simulink model "WarehouseFleetSim"  (R2024b)
settings: Solver=ode4  StartTime=0.0  StopTime=inf  FixedStep=0.02  RelTol=1e-3
StopFcn:
  | try, fleetVisionStep('close'); catch, end; try, phase3('stopped'); catch, end
model workspace (MAT data in the model file):
  HomePose1 = [-20 7.3 0]
  HomePose2 = [-20 3.6 0]
  HomePose3 = [-20 11 0]
  HomePose4 = [-24.5 3.6 0]
  HomePose5 = [-24.5 7.3 0]
  HomePose6 = [-24.5 11 0]
  Zero = 0
  gen3 : robotics.RigidBodyTree (value not decoded)
  qStow = [0; 0; 0.261799387799; 3.14159265359; -2.26892802759; 0; 0.959931088597; 1.57079632679]
undefined symbols (not defined in the file or in its folder): Actor, setupFleetScene, Sim3dSensor, World
libraries: sim3dlib x128, sim3dcameralib x7, robotmobilelib x6, robotsim3dlib x6
(part 3 of 4)

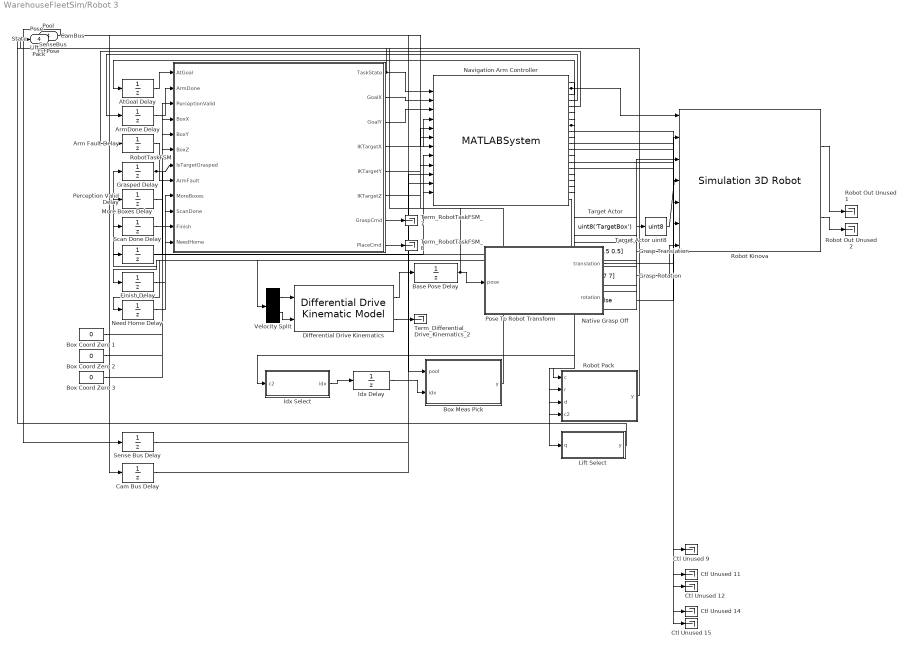
== system WarehouseFleetSim/Robot 3 ==
  Pool : Inport
  EstPose : Inport  Port=2
  SenseBus : Inport  Port=3
  CamBus : Inport  Port=4
  Arm Fault Delay : UnitDelay  InitialCondition=false  SampleTime=0.02  HasFrameUpgradeWarning=on
  ArmDone Delay : UnitDelay  InitialCondition=false  SampleTime=0.02  HasFrameUpgradeWarning=on
  AtGoal Delay : UnitDelay  InitialCondition=false  SampleTime=0.02  HasFrameUpgradeWarning=on
  Base Pose Delay : UnitDelay  InitialCondition=HomePose3  SampleTime=0.02  HasFrameUpgradeWarning=on
  Box Coord Zero 1 : Constant  Value=0  OutDataTypeStr=double
  Box Coord Zero 2 : Constant  Value=0  OutDataTypeStr=double
  Box Coord Zero 3 : Constant  Value=0  OutDataTypeStr=double
  Box Meas Pick : MATLAB Function  TreatAsAtomicUnit=on
  Cam Bus Delay : UnitDelay  InitialCondition=zeros(1,8)  SampleTime=0.02  HasFrameUpgradeWarning=on
  Ctl Unused {9,11..12,14..15} (5 alike) : Terminator
  Differential Drive Kinematics : robotmobilelib/Differential Drive Kinematic Model  VehicleInputs=Vehicle Speed & Heading Angular Velocity  WheelRadius=0.05  WheelSpeedRange=[-inf inf]  TrackWidth=0.2  InitialState=HomePose3  SimulateUsing=Interpreted execution
  Finish Delay : UnitDelay  InitialCondition=false  SampleTime=0.02  HasFrameUpgradeWarning=on
  Grasp Rotation : Constant  Value=[7 7 7]
  Grasp Translation : Constant  Value=[0.5 0.5 0.5]
  Grasped Delay : UnitDelay  InitialCondition=false  SampleTime=0.02  HasFrameUpgradeWarning=on
  Idx Delay : UnitDelay  SampleTime=0.02  HasFrameUpgradeWarning=on
  Idx Select : MATLAB Function  TreatAsAtomicUnit=on
  Lift Select : MATLAB Function  TreatAsAtomicUnit=on
  More Boxes Delay : UnitDelay  InitialCondition=false  SampleTime=0.02  HasFrameUpgradeWarning=on
  Native Grasp Off : Constant  Value=false  OutDataTypeStr=boolean
  Navigation Arm Controller : MATLABSystem  System=WarehouseRobotControlSystemV23  SampleTime=0.02  RobotId=3  SimulateUsing=Interpreted execution
      mask Type: WarehouseRobotControlSystemV23
      mask Display:
      | disp('WarehouseRobotControlSystemV23');
      | port_label('input',1,'state');
      | port_label('input',2,'~');
      | port_label('input',3,'~');
      | port_label('input',4,'~');
      | port_label('input',5,'~');
      | port_label('input',6,'~');
      | port_label('input',7,'basePose');
      | port_label('input',8,'isTargetGrasped');
      | port_label('input',9,'boxMeas');
      | port_label('input',10,'senseBus');
      | port_label('input',11,'camBus');
      | port_label('input',12,'truePose');
      | port_label('output',1,'velocity');
      | port_label('output',2,'config');
      | port_label('output',3,'atGoal');
      | port_label('output',4,'armDone');
      | port_label('output',5,'armFault');
      | port_label('output',6,'vacuum');
      | port_label('output',7,'c1');
      | port_label('output',8,'c2');
      | port_label('output',9,'c3');
      | port_label('output',10,'r1');
      | port_label('output',11,'r2');
      | port_label('output',12,'r3');
      | port_label('output',13,'d1');
      | port_label('output',14,'d2');
      | port_label('output',15,'d3');
      | port_label('output',16,'percValid');
      | port_label('output',17,'moreBoxes');
      | port_label('output',18,'scanDone');
      | port_label('output',19,'finish');
      | port_label('output',20,'needHome');
  Need Home Delay : UnitDelay  InitialCondition=false  SampleTime=0.02  HasFrameUpgradeWarning=on
  Perception Valid Delay : UnitDelay  InitialCondition=false  SampleTime=0.02  HasFrameUpgradeWarning=on
  Pose To Robot Transform : MATLAB Function  TreatAsAtomicUnit=on
  Robot Kinova : robotsim3dlib/Simulation 3D Robot  Priority=2  actorInputType=RigidBodyTree Object  RigidBodyTree=gen3  ActorName=Ro3Kinova  existActorChekBox=off  initialTrans=[0 0 0]  initialRot=[0 0 0]  initialConfig=qStow  EndEffector=ToolTip  eeOffsetInpChekBox=off  eeTargetTrans=[-0.04 0 0.245]  eeTargetRot=[0 1.2217 3.1416]  enableRegionGraspChekBox=on  regionGraspInpChekBox=on  eeTargTransDiff=[0.2 0.2 0.2]  eeTargRotDiff=[0 0 0]  inpConfEnbVal=on  inpGraspEnbVal=on  inpTransEnbVal=on  outConfEnbVal=on  outGraspEnbVal=on  outTransEnbVal=off  SampleTime=0.02  ActorType=SimulinkVehicle  ID=C  aMode=6  ActorTag=Ro3Kinova  Mesh=RigidBodyTree
  Robot Out Unused 1 : Terminator
  Robot Out Unused 2 : Terminator
  Robot Pack : MATLAB Function  TreatAsAtomicUnit=on
  RobotTaskFSM : Stateflow chart  TreatAsAtomicUnit=on
  Scan Done Delay : UnitDelay  InitialCondition=false  SampleTime=0.02  HasFrameUpgradeWarning=on
  Sense Bus Delay : UnitDelay  InitialCondition=zeros(1,8)  SampleTime=0.02  HasFrameUpgradeWarning=on
  Target Actor : Constant  Value=uint8('TargetBox')  OutDataTypeStr=uint8
  Target Actor uint8 : DataTypeConversion  OutDataTypeStr=uint8  SaturateOnIntegerOverflow=off  RndMeth=Floor
  Term_Differential_Drive_Kinematics_2 : Terminator
  Term_RobotTaskFSM_7 : Terminator
  Term_RobotTaskFSM_8 : Terminator
  Velocity Split : Demux  Outputs=2
  Pose : Outport
  Pack : Outport  Port=2
  Lift : Outport  Port=3
  State : Outport  Port=4
  wires:
  Navigation Arm Controller/3 -> AtGoal Delay/1
  AtGoal Delay/1 -> RobotTaskFSM/1(AtGoal)
  Navigation Arm Controller/4 -> ArmDone Delay/1
  ArmDone Delay/1 -> RobotTaskFSM/2(ArmDone)
  Navigation Arm Controller/5 -> Arm Fault Delay/1
  Arm Fault Delay/1 -> RobotTaskFSM/8(ArmFault)
  Navigation Arm Controller/6 -> Grasped Delay/1
  Grasped Delay/1 -> RobotTaskFSM/7(IsTargetGrasped), Navigation Arm Controller/8
  Navigation Arm Controller/16 -> Perception Valid Delay/1
  Perception Valid Delay/1 -> RobotTaskFSM/3(PerceptionValid)
  Navigation Arm Controller/17 -> More Boxes Delay/1
  More Boxes Delay/1 -> RobotTaskFSM/9(MoreBoxes)
  Navigation Arm Controller/18 -> Scan Done Delay/1
  Scan Done Delay/1 -> RobotTaskFSM/10(ScanDone)
  Navigation Arm Controller/19 -> Finish Delay/1
  Finish Delay/1 -> RobotTaskFSM/11(Finish)
  Navigation Arm Controller/20 -> Need Home Delay/1
  Need Home Delay/1 -> RobotTaskFSM/12(NeedHome)
  Box Coord Zero 1/1 -> RobotTaskFSM/4(BoxX)
  Box Coord Zero 2/1 -> RobotTaskFSM/5(BoxY)
  Box Coord Zero 3/1 -> RobotTaskFSM/6(BoxZ)
  RobotTaskFSM/1(TaskState) -> Navigation Arm Controller/1, State/1
  RobotTaskFSM/2(GoalX) -> Navigation Arm Controller/2
  RobotTaskFSM/3(GoalY) -> Navigation Arm Controller/3
  RobotTaskFSM/4(IKTargetX) -> Navigation Arm Controller/4
  RobotTaskFSM/5(IKTargetY) -> Navigation Arm Controller/5
  RobotTaskFSM/6(IKTargetZ) -> Navigation Arm Controller/6
  EstPose/1 -> Navigation Arm Controller/7
  SenseBus/1 -> Sense Bus Delay/1
  Sense Bus Delay/1 -> Navigation Arm Controller/10
  CamBus/1 -> Cam Bus Delay/1
  Cam Bus Delay/1 -> Navigation Arm Controller/11
  Base Pose Delay/1 -> Navigation Arm Controller/12, Pose/1, Pose To Robot Transform/1(pose)
  Navigation Arm Controller/8 -> Idx Select/1(c2), Robot Pack/4(c2)
  Idx Select/1(idx) -> Idx Delay/1
  Idx Delay/1 -> Box Meas Pick/2(idx)
  Pool/1 -> Box Meas Pick/1(pool)
  Box Meas Pick/1(y) -> Navigation Arm Controller/9
  Navigation Arm Controller/7 -> Robot Pack/1(c)
  Navigation Arm Controller/10 -> Robot Pack/2(r)
  Navigation Arm Controller/13 -> Robot Pack/3(d)
  Robot Pack/1(y) -> Pack/1
  Navigation Arm Controller/2 -> Lift Select/1(q), Robot Kinova/1
  Lift Select/1(y) -> Lift/1
  Navigation Arm Controller/9 -> Ctl Unused 9/1
  Navigation Arm Controller/11 -> Ctl Unused 11/1
  Navigation Arm Controller/12 -> Ctl Unused 12/1
  Navigation Arm Controller/14 -> Ctl Unused 14/1
  Navigation Arm Controller/15 -> Ctl Unused 15/1
  Navigation Arm Controller/1 -> Velocity Split/1
  Velocity Split/1 -> Differential Drive Kinematics/1
  Velocity Split/2 -> Differential Drive Kinematics/2
  Differential Drive Kinematics/1 -> Base Pose Delay/1
  Target Actor/1 -> Target Actor uint8/1
  Pose To Robot Transform/1(translation) -> Robot Kinova/2
  Pose To Robot Transform/2(rotation) -> Robot Kinova/3
  Target Actor uint8/1 -> Robot Kinova/4
  Native Grasp Off/1 -> Robot Kinova/5
  Grasp Translation/1 -> Robot Kinova/6
  Grasp Rotation/1 -> Robot Kinova/7
  Robot Kinova/1 -> Robot Out Unused 1/1
  Robot Kinova/2 -> Robot Out Unused 2/1
  Differential Drive Kinematics/2 -> Term_Differential_Drive_Kinematics_2/1
  RobotTaskFSM/7(GraspCmd) -> Term_RobotTaskFSM_7/1
  RobotTaskFSM/8(PlaceCmd) -> Term_RobotTaskFSM_8/1

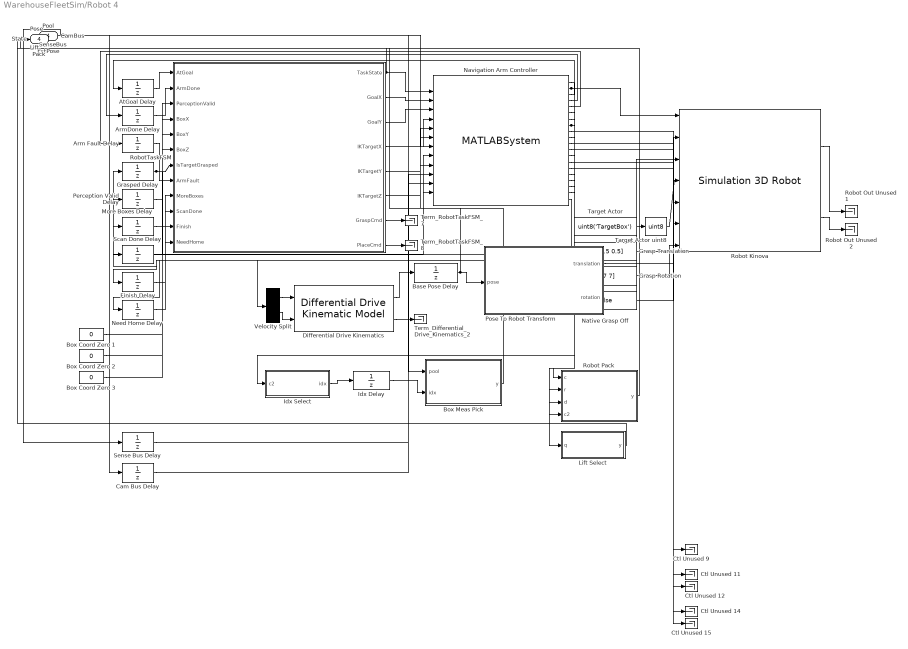
== system WarehouseFleetSim/Robot 4 ==
  Pool : Inport
  EstPose : Inport  Port=2
  SenseBus : Inport  Port=3
  CamBus : Inport  Port=4
  Arm Fault Delay : UnitDelay  InitialCondition=false  SampleTime=0.02  HasFrameUpgradeWarning=on
  ArmDone Delay : UnitDelay  InitialCondition=false  SampleTime=0.02  HasFrameUpgradeWarning=on
  AtGoal Delay : UnitDelay  InitialCondition=false  SampleTime=0.02  HasFrameUpgradeWarning=on
  Base Pose Delay : UnitDelay  InitialCondition=HomePose4  SampleTime=0.02  HasFrameUpgradeWarning=on
  Box Coord Zero 1 : Constant  Value=0  OutDataTypeStr=double
  Box Coord Zero 2 : Constant  Value=0  OutDataTypeStr=double
  Box Coord Zero 3 : Constant  Value=0  OutDataTypeStr=double
  Box Meas Pick : MATLAB Function  TreatAsAtomicUnit=on
  Cam Bus Delay : UnitDelay  InitialCondition=zeros(1,8)  SampleTime=0.02  HasFrameUpgradeWarning=on
  Ctl Unused {9,11..12,14..15} (5 alike) : Terminator
  Differential Drive Kinematics : robotmobilelib/Differential Drive Kinematic Model  VehicleInputs=Vehicle Speed & Heading Angular Velocity  WheelRadius=0.05  WheelSpeedRange=[-inf inf]  TrackWidth=0.2  InitialState=HomePose4  SimulateUsing=Interpreted execution
  Finish Delay : UnitDelay  InitialCondition=false  SampleTime=0.02  HasFrameUpgradeWarning=on
  Grasp Rotation : Constant  Value=[7 7 7]
  Grasp Translation : Constant  Value=[0.5 0.5 0.5]
  Grasped Delay : UnitDelay  InitialCondition=false  SampleTime=0.02  HasFrameUpgradeWarning=on
  Idx Delay : UnitDelay  SampleTime=0.02  HasFrameUpgradeWarning=on
  Idx Select : MATLAB Function  TreatAsAtomicUnit=on
  Lift Select : MATLAB Function  TreatAsAtomicUnit=on
  More Boxes Delay : UnitDelay  InitialCondition=false  SampleTime=0.02  HasFrameUpgradeWarning=on
  Native Grasp Off : Constant  Value=false  OutDataTypeStr=boolean
  Navigation Arm Controller : MATLABSystem  System=WarehouseRobotControlSystemV23  SampleTime=0.02  RobotId=4  SimulateUsing=Interpreted execution
      mask Type: WarehouseRobotControlSystemV23
      mask Display:
      | disp('WarehouseRobotControlSystemV23');
      | port_label('input',1,'state');
      | port_label('input',2,'~');
      | port_label('input',3,'~');
      | port_label('input',4,'~');
      | port_label('input',5,'~');
      | port_label('input',6,'~');
      | port_label('input',7,'basePose');
      | port_label('input',8,'isTargetGrasped');
      | port_label('input',9,'boxMeas');
      | port_label('input',10,'senseBus');
      | port_label('input',11,'camBus');
      | port_label('input',12,'truePose');
      | port_label('output',1,'velocity');
      | port_label('output',2,'config');
      | port_label('output',3,'atGoal');
      | port_label('output',4,'armDone');
      | port_label('output',5,'armFault');
      | port_label('output',6,'vacuum');
      | port_label('output',7,'c1');
      | port_label('output',8,'c2');
      | port_label('output',9,'c3');
      | port_label('output',10,'r1');
      | port_label('output',11,'r2');
      | port_label('output',12,'r3');
      | port_label('output',13,'d1');
      | port_label('output',14,'d2');
      | port_label('output',15,'d3');
      | port_label('output',16,'percValid');
      | port_label('output',17,'moreBoxes');
      | port_label('output',18,'scanDone');
      | port_label('output',19,'finish');
      | port_label('output',20,'needHome');
  Need Home Delay : UnitDelay  InitialCondition=false  SampleTime=0.02  HasFrameUpgradeWarning=on
  Perception Valid Delay : UnitDelay  InitialCondition=false  SampleTime=0.02  HasFrameUpgradeWarning=on
  Pose To Robot Transform : MATLAB Function  TreatAsAtomicUnit=on
  Robot Kinova : robotsim3dlib/Simulation 3D Robot  Priority=2  actorInputType=RigidBodyTree Object  RigidBodyTree=gen3  ActorName=Ro4Kinova  existActorChekBox=off  initialTrans=[0 0 0]  initialRot=[0 0 0]  initialConfig=qStow  EndEffector=ToolTip  eeOffsetInpChekBox=off  eeTargetTrans=[-0.04 0 0.245]  eeTargetRot=[0 1.2217 3.1416]  enableRegionGraspChekBox=on  regionGraspInpChekBox=on  eeTargTransDiff=[0.2 0.2 0.2]  eeTargRotDiff=[0 0 0]  inpConfEnbVal=on  inpGraspEnbVal=on  inpTransEnbVal=on  outConfEnbVal=on  outGraspEnbVal=on  outTransEnbVal=off  SampleTime=0.02  ActorType=SimulinkVehicle  ID=C  aMode=6  ActorTag=Ro4Kinova  Mesh=RigidBodyTree
  Robot Out Unused 1 : Terminator
  Robot Out Unused 2 : Terminator
  Robot Pack : MATLAB Function  TreatAsAtomicUnit=on
  RobotTaskFSM : Stateflow chart  TreatAsAtomicUnit=on
  Scan Done Delay : UnitDelay  InitialCondition=false  SampleTime=0.02  HasFrameUpgradeWarning=on
  Sense Bus Delay : UnitDelay  InitialCondition=zeros(1,8)  SampleTime=0.02  HasFrameUpgradeWarning=on
  Target Actor : Constant  Value=uint8('TargetBox')  OutDataTypeStr=uint8
  Target Actor uint8 : DataTypeConversion  OutDataTypeStr=uint8  SaturateOnIntegerOverflow=off  RndMeth=Floor
  Term_Differential_Drive_Kinematics_2 : Terminator
  Term_RobotTaskFSM_7 : Terminator
  Term_RobotTaskFSM_8 : Terminator
  Velocity Split : Demux  Outputs=2
  Pose : Outport
  Pack : Outport  Port=2
  Lift : Outport  Port=3
  State : Outport  Port=4
  wires:
  Navigation Arm Controller/3 -> AtGoal Delay/1
  AtGoal Delay/1 -> RobotTaskFSM/1(AtGoal)
  Navigation Arm Controller/4 -> ArmDone Delay/1
  ArmDone Delay/1 -> RobotTaskFSM/2(ArmDone)
  Navigation Arm Controller/5 -> Arm Fault Delay/1
  Arm Fault Delay/1 -> RobotTaskFSM/8(ArmFault)
  Navigation Arm Controller/6 -> Grasped Delay/1
  Grasped Delay/1 -> RobotTaskFSM/7(IsTargetGrasped), Navigation Arm Controller/8
  Navigation Arm Controller/16 -> Perception Valid Delay/1
  Perception Valid Delay/1 -> RobotTaskFSM/3(PerceptionValid)
  Navigation Arm Controller/17 -> More Boxes Delay/1
  More Boxes Delay/1 -> RobotTaskFSM/9(MoreBoxes)
  Navigation Arm Controller/18 -> Scan Done Delay/1
  Scan Done Delay/1 -> RobotTaskFSM/10(ScanDone)
  Navigation Arm Controller/19 -> Finish Delay/1
  Finish Delay/1 -> RobotTaskFSM/11(Finish)
  Navigation Arm Controller/20 -> Need Home Delay/1
  Need Home Delay/1 -> RobotTaskFSM/12(NeedHome)
  Box Coord Zero 1/1 -> RobotTaskFSM/4(BoxX)
  Box Coord Zero 2/1 -> RobotTaskFSM/5(BoxY)
  Box Coord Zero 3/1 -> RobotTaskFSM/6(BoxZ)
  RobotTaskFSM/1(TaskState) -> Navigation Arm Controller/1, State/1
  RobotTaskFSM/2(GoalX) -> Navigation Arm Controller/2
  RobotTaskFSM/3(GoalY) -> Navigation Arm Controller/3
  RobotTaskFSM/4(IKTargetX) -> Navigation Arm Controller/4
  RobotTaskFSM/5(IKTargetY) -> Navigation Arm Controller/5
  RobotTaskFSM/6(IKTargetZ) -> Navigation Arm Controller/6
  EstPose/1 -> Navigation Arm Controller/7
  SenseBus/1 -> Sense Bus Delay/1
  Sense Bus Delay/1 -> Navigation Arm Controller/10
  CamBus/1 -> Cam Bus Delay/1
  Cam Bus Delay/1 -> Navigation Arm Controller/11
  Base Pose Delay/1 -> Navigation Arm Controller/12, Pose/1, Pose To Robot Transform/1(pose)
  Navigation Arm Controller/8 -> Idx Select/1(c2), Robot Pack/4(c2)
  Idx Select/1(idx) -> Idx Delay/1
  Idx Delay/1 -> Box Meas Pick/2(idx)
  Pool/1 -> Box Meas Pick/1(pool)
  Box Meas Pick/1(y) -> Navigation Arm Controller/9
  Navigation Arm Controller/7 -> Robot Pack/1(c)
  Navigation Arm Controller/10 -> Robot Pack/2(r)
  Navigation Arm Controller/13 -> Robot Pack/3(d)
  Robot Pack/1(y) -> Pack/1
  Navigation Arm Controller/2 -> Lift Select/1(q), Robot Kinova/1
  Lift Select/1(y) -> Lift/1
  Navigation Arm Controller/9 -> Ctl Unused 9/1
  Navigation Arm Controller/11 -> Ctl Unused 11/1
  Navigation Arm Controller/12 -> Ctl Unused 12/1
  Navigation Arm Controller/14 -> Ctl Unused 14/1
  Navigation Arm Controller/15 -> Ctl Unused 15/1
  Navigation Arm Controller/1 -> Velocity Split/1
  Velocity Split/1 -> Differential Drive Kinematics/1
  Velocity Split/2 -> Differential Drive Kinematics/2
  Differential Drive Kinematics/1 -> Base Pose Delay/1
  Target Actor/1 -> Target Actor uint8/1
  Pose To Robot Transform/1(translation) -> Robot Kinova/2
  Pose To Robot Transform/2(rotation) -> Robot Kinova/3
  Target Actor uint8/1 -> Robot Kinova/4
  Native Grasp Off/1 -> Robot Kinova/5
  Grasp Translation/1 -> Robot Kinova/6
  Grasp Rotation/1 -> Robot Kinova/7
  Robot Kinova/1 -> Robot Out Unused 1/1
  Robot Kinova/2 -> Robot Out Unused 2/1
  Differential Drive Kinematics/2 -> Term_Differential_Drive_Kinematics_2/1
  RobotTaskFSM/7(GraspCmd) -> Term_RobotTaskFSM_7/1
  RobotTaskFSM/8(PlaceCmd) -> Term_RobotTaskFSM_8/1

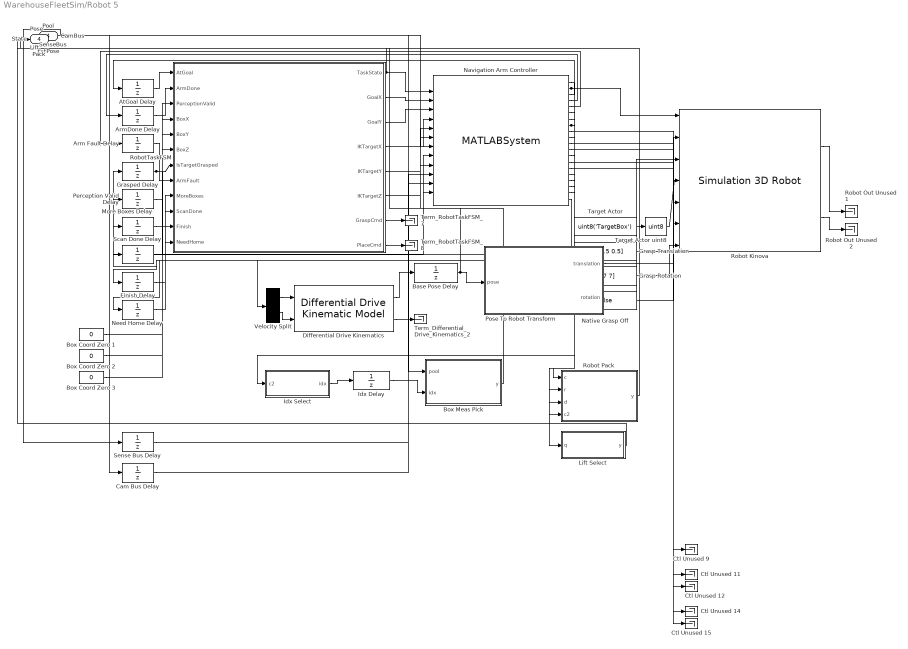
== system WarehouseFleetSim/Robot 5 ==
  Pool : Inport
  EstPose : Inport  Port=2
  SenseBus : Inport  Port=3
  CamBus : Inport  Port=4
  Arm Fault Delay : UnitDelay  InitialCondition=false  SampleTime=0.02  HasFrameUpgradeWarning=on
  ArmDone Delay : UnitDelay  InitialCondition=false  SampleTime=0.02  HasFrameUpgradeWarning=on
  AtGoal Delay : UnitDelay  InitialCondition=false  SampleTime=0.02  HasFrameUpgradeWarning=on
  Base Pose Delay : UnitDelay  InitialCondition=HomePose5  SampleTime=0.02  HasFrameUpgradeWarning=on
  Box Coord Zero 1 : Constant  Value=0  OutDataTypeStr=double
  Box Coord Zero 2 : Constant  Value=0  OutDataTypeStr=double
  Box Coord Zero 3 : Constant  Value=0  OutDataTypeStr=double
  Box Meas Pick : MATLAB Function  TreatAsAtomicUnit=on
  Cam Bus Delay : UnitDelay  InitialCondition=zeros(1,8)  SampleTime=0.02  HasFrameUpgradeWarning=on
  Ctl Unused {9,11..12,14..15} (5 alike) : Terminator
  Differential Drive Kinematics : robotmobilelib/Differential Drive Kinematic Model  VehicleInputs=Vehicle Speed & Heading Angular Velocity  WheelRadius=0.05  WheelSpeedRange=[-inf inf]  TrackWidth=0.2  InitialState=HomePose5  SimulateUsing=Interpreted execution
  Finish Delay : UnitDelay  InitialCondition=false  SampleTime=0.02  HasFrameUpgradeWarning=on
  Grasp Rotation : Constant  Value=[7 7 7]
  Grasp Translation : Constant  Value=[0.5 0.5 0.5]
  Grasped Delay : UnitDelay  InitialCondition=false  SampleTime=0.02  HasFrameUpgradeWarning=on
  Idx Delay : UnitDelay  SampleTime=0.02  HasFrameUpgradeWarning=on
  Idx Select : MATLAB Function  TreatAsAtomicUnit=on
  Lift Select : MATLAB Function  TreatAsAtomicUnit=on
  More Boxes Delay : UnitDelay  InitialCondition=false  SampleTime=0.02  HasFrameUpgradeWarning=on
  Native Grasp Off : Constant  Value=false  OutDataTypeStr=boolean
  Navigation Arm Controller : MATLABSystem  System=WarehouseRobotControlSystemV23  SampleTime=0.02  RobotId=5  SimulateUsing=Interpreted execution
      mask Type: WarehouseRobotControlSystemV23
      mask Display:
      | disp('WarehouseRobotControlSystemV23');
      | port_label('input',1,'state');
      | port_label('input',2,'~');
      | port_label('input',3,'~');
      | port_label('input',4,'~');
      | port_label('input',5,'~');
      | port_label('input',6,'~');
      | port_label('input',7,'basePose');
      | port_label('input',8,'isTargetGrasped');
      | port_label('input',9,'boxMeas');
      | port_label('input',10,'senseBus');
      | port_label('input',11,'camBus');
      | port_label('input',12,'truePose');
      | port_label('output',1,'velocity');
      | port_label('output',2,'config');
      | port_label('output',3,'atGoal');
      | port_label('output',4,'armDone');
      | port_label('output',5,'armFault');
      | port_label('output',6,'vacuum');
      | port_label('output',7,'c1');
      | port_label('output',8,'c2');
      | port_label('output',9,'c3');
      | port_label('output',10,'r1');
      | port_label('output',11,'r2');
      | port_label('output',12,'r3');
      | port_label('output',13,'d1');
      | port_label('output',14,'d2');
      | port_label('output',15,'d3');
      | port_label('output',16,'percValid');
      | port_label('output',17,'moreBoxes');
      | port_label('output',18,'scanDone');
      | port_label('output',19,'finish');
      | port_label('output',20,'needHome');
  Need Home Delay : UnitDelay  InitialCondition=false  SampleTime=0.02  HasFrameUpgradeWarning=on
  Perception Valid Delay : UnitDelay  InitialCondition=false  SampleTime=0.02  HasFrameUpgradeWarning=on
  Pose To Robot Transform : MATLAB Function  TreatAsAtomicUnit=on
  Robot Kinova : robotsim3dlib/Simulation 3D Robot  Priority=2  actorInputType=RigidBodyTree Object  RigidBodyTree=gen3  ActorName=Ro5Kinova  existActorChekBox=off  initialTrans=[0 0 0]  initialRot=[0 0 0]  initialConfig=qStow  EndEffector=ToolTip  eeOffsetInpChekBox=off  eeTargetTrans=[-0.04 0 0.245]  eeTargetRot=[0 1.2217 3.1416]  enableRegionGraspChekBox=on  regionGraspInpChekBox=on  eeTargTransDiff=[0.2 0.2 0.2]  eeTargRotDiff=[0 0 0]  inpConfEnbVal=on  inpGraspEnbVal=on  inpTransEnbVal=on  outConfEnbVal=on  outGraspEnbVal=on  outTransEnbVal=off  SampleTime=0.02  ActorType=SimulinkVehicle  ID=C  aMode=6  ActorTag=Ro5Kinova  Mesh=RigidBodyTree
  Robot Out Unused 1 : Terminator
  Robot Out Unused 2 : Terminator
  Robot Pack : MATLAB Function  TreatAsAtomicUnit=on
  RobotTaskFSM : Stateflow chart  TreatAsAtomicUnit=on
  Scan Done Delay : UnitDelay  InitialCondition=false  SampleTime=0.02  HasFrameUpgradeWarning=on
  Sense Bus Delay : UnitDelay  InitialCondition=zeros(1,8)  SampleTime=0.02  HasFrameUpgradeWarning=on
  Target Actor : Constant  Value=uint8('TargetBox')  OutDataTypeStr=uint8
  Target Actor uint8 : DataTypeConversion  OutDataTypeStr=uint8  SaturateOnIntegerOverflow=off  RndMeth=Floor
  Term_Differential_Drive_Kinematics_2 : Terminator
  Term_RobotTaskFSM_7 : Terminator
  Term_RobotTaskFSM_8 : Terminator
  Velocity Split : Demux  Outputs=2
  Pose : Outport
  Pack : Outport  Port=2
  Lift : Outport  Port=3
  State : Outport  Port=4
  wires:
  Navigation Arm Controller/3 -> AtGoal Delay/1
  AtGoal Delay/1 -> RobotTaskFSM/1(AtGoal)
  Navigation Arm Controller/4 -> ArmDone Delay/1
  ArmDone Delay/1 -> RobotTaskFSM/2(ArmDone)
  Navigation Arm Controller/5 -> Arm Fault Delay/1
  Arm Fault Delay/1 -> RobotTaskFSM/8(ArmFault)
  Navigation Arm Controller/6 -> Grasped Delay/1
  Grasped Delay/1 -> RobotTaskFSM/7(IsTargetGrasped), Navigation Arm Controller/8
  Navigation Arm Controller/16 -> Perception Valid Delay/1
  Perception Valid Delay/1 -> RobotTaskFSM/3(PerceptionValid)
  Navigation Arm Controller/17 -> More Boxes Delay/1
  More Boxes Delay/1 -> RobotTaskFSM/9(MoreBoxes)
  Navigation Arm Controller/18 -> Scan Done Delay/1
  Scan Done Delay/1 -> RobotTaskFSM/10(ScanDone)
  Navigation Arm Controller/19 -> Finish Delay/1
  Finish Delay/1 -> RobotTaskFSM/11(Finish)
  Navigation Arm Controller/20 -> Need Home Delay/1
  Need Home Delay/1 -> RobotTaskFSM/12(NeedHome)
  Box Coord Zero 1/1 -> RobotTaskFSM/4(BoxX)
  Box Coord Zero 2/1 -> RobotTaskFSM/5(BoxY)
  Box Coord Zero 3/1 -> RobotTaskFSM/6(BoxZ)
  RobotTaskFSM/1(TaskState) -> Navigation Arm Controller/1, State/1
  RobotTaskFSM/2(GoalX) -> Navigation Arm Controller/2
  RobotTaskFSM/3(GoalY) -> Navigation Arm Controller/3
  RobotTaskFSM/4(IKTargetX) -> Navigation Arm Controller/4
  RobotTaskFSM/5(IKTargetY) -> Navigation Arm Controller/5
  RobotTaskFSM/6(IKTargetZ) -> Navigation Arm Controller/6
  EstPose/1 -> Navigation Arm Controller/7
  SenseBus/1 -> Sense Bus Delay/1
  Sense Bus Delay/1 -> Navigation Arm Controller/10
  CamBus/1 -> Cam Bus Delay/1
  Cam Bus Delay/1 -> Navigation Arm Controller/11
  Base Pose Delay/1 -> Navigation Arm Controller/12, Pose/1, Pose To Robot Transform/1(pose)
  Navigation Arm Controller/8 -> Idx Select/1(c2), Robot Pack/4(c2)
  Idx Select/1(idx) -> Idx Delay/1
  Idx Delay/1 -> Box Meas Pick/2(idx)
  Pool/1 -> Box Meas Pick/1(pool)
  Box Meas Pick/1(y) -> Navigation Arm Controller/9
  Navigation Arm Controller/7 -> Robot Pack/1(c)
  Navigation Arm Controller/10 -> Robot Pack/2(r)
  Navigation Arm Controller/13 -> Robot Pack/3(d)
  Robot Pack/1(y) -> Pack/1
  Navigation Arm Controller/2 -> Lift Select/1(q), Robot Kinova/1
  Lift Select/1(y) -> Lift/1
  Navigation Arm Controller/9 -> Ctl Unused 9/1
  Navigation Arm Controller/11 -> Ctl Unused 11/1
  Navigation Arm Controller/12 -> Ctl Unused 12/1
  Navigation Arm Controller/14 -> Ctl Unused 14/1
  Navigation Arm Controller/15 -> Ctl Unused 15/1
  Navigation Arm Controller/1 -> Velocity Split/1
  Velocity Split/1 -> Differential Drive Kinematics/1
  Velocity Split/2 -> Differential Drive Kinematics/2
  Differential Drive Kinematics/1 -> Base Pose Delay/1
  Target Actor/1 -> Target Actor uint8/1
  Pose To Robot Transform/1(translation) -> Robot Kinova/2
  Pose To Robot Transform/2(rotation) -> Robot Kinova/3
  Target Actor uint8/1 -> Robot Kinova/4
  Native Grasp Off/1 -> Robot Kinova/5
  Grasp Translation/1 -> Robot Kinova/6
  Grasp Rotation/1 -> Robot Kinova/7
  Robot Kinova/1 -> Robot Out Unused 1/1
  Robot Kinova/2 -> Robot Out Unused 2/1
  Differential Drive Kinematics/2 -> Term_Differential_Drive_Kinematics_2/1
  RobotTaskFSM/7(GraspCmd) -> Term_RobotTaskFSM_7/1
  RobotTaskFSM/8(PlaceCmd) -> Term_RobotTaskFSM_8/1

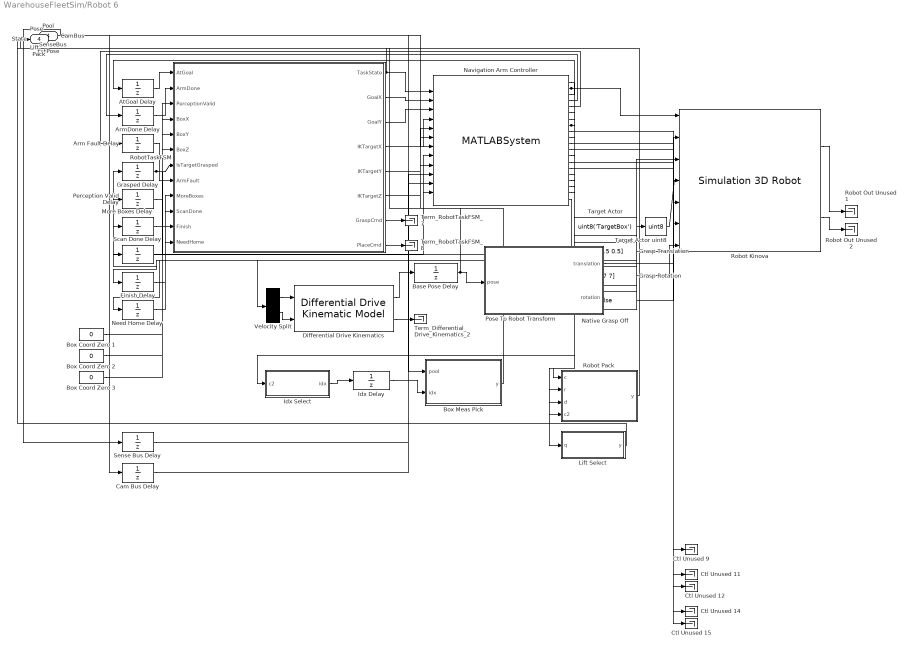
== system WarehouseFleetSim/Robot 6 ==
  Pool : Inport
  EstPose : Inport  Port=2
  SenseBus : Inport  Port=3
  CamBus : Inport  Port=4
  Arm Fault Delay : UnitDelay  InitialCondition=false  SampleTime=0.02  HasFrameUpgradeWarning=on
  ArmDone Delay : UnitDelay  InitialCondition=false  SampleTime=0.02  HasFrameUpgradeWarning=on
  AtGoal Delay : UnitDelay  InitialCondition=false  SampleTime=0.02  HasFrameUpgradeWarning=on
  Base Pose Delay : UnitDelay  InitialCondition=HomePose6  SampleTime=0.02  HasFrameUpgradeWarning=on
  Box Coord Zero 1 : Constant  Value=0  OutDataTypeStr=double
  Box Coord Zero 2 : Constant  Value=0  OutDataTypeStr=double
  Box Coord Zero 3 : Constant  Value=0  OutDataTypeStr=double
  Box Meas Pick : MATLAB Function  TreatAsAtomicUnit=on
  Cam Bus Delay : UnitDelay  InitialCondition=zeros(1,8)  SampleTime=0.02  HasFrameUpgradeWarning=on
  Ctl Unused {9,11..12,14..15} (5 alike) : Terminator
  Differential Drive Kinematics : robotmobilelib/Differential Drive Kinematic Model  VehicleInputs=Vehicle Speed & Heading Angular Velocity  WheelRadius=0.05  WheelSpeedRange=[-inf inf]  TrackWidth=0.2  InitialState=HomePose6  SimulateUsing=Interpreted execution
  Finish Delay : UnitDelay  InitialCondition=false  SampleTime=0.02  HasFrameUpgradeWarning=on
  Grasp Rotation : Constant  Value=[7 7 7]
  Grasp Translation : Constant  Value=[0.5 0.5 0.5]
  Grasped Delay : UnitDelay  InitialCondition=false  SampleTime=0.02  HasFrameUpgradeWarning=on
  Idx Delay : UnitDelay  SampleTime=0.02  HasFrameUpgradeWarning=on
  Idx Select : MATLAB Function  TreatAsAtomicUnit=on
  Lift Select : MATLAB Function  TreatAsAtomicUnit=on
  More Boxes Delay : UnitDelay  InitialCondition=false  SampleTime=0.02  HasFrameUpgradeWarning=on
  Native Grasp Off : Constant  Value=false  OutDataTypeStr=boolean
  Navigation Arm Controller : MATLABSystem  System=WarehouseRobotControlSystemV23  SampleTime=0.02  RobotId=6  SimulateUsing=Interpreted execution
      mask Type: WarehouseRobotControlSystemV23
      mask Display:
      | disp('WarehouseRobotControlSystemV23');
      | port_label('input',1,'state');
      | port_label('input',2,'~');
      | port_label('input',3,'~');
      | port_label('input',4,'~');
      | port_label('input',5,'~');
      | port_label('input',6,'~');
      | port_label('input',7,'basePose');
      | port_label('input',8,'isTargetGrasped');
      | port_label('input',9,'boxMeas');
      | port_label('input',10,'senseBus');
      | port_label('input',11,'camBus');
      | port_label('input',12,'truePose');
      | port_label('output',1,'velocity');
      | port_label('output',2,'config');
      | port_label('output',3,'atGoal');
      | port_label('output',4,'armDone');
      | port_label('output',5,'armFault');
      | port_label('output',6,'vacuum');
      | port_label('output',7,'c1');
      | port_label('output',8,'c2');
      | port_label('output',9,'c3');
      | port_label('output',10,'r1');
      | port_label('output',11,'r2');
      | port_label('output',12,'r3');
      | port_label('output',13,'d1');
      | port_label('output',14,'d2');
      | port_label('output',15,'d3');
      | port_label('output',16,'percValid');
      | port_label('output',17,'moreBoxes');
      | port_label('output',18,'scanDone');
      | port_label('output',19,'finish');
      | port_label('output',20,'needHome');
  Need Home Delay : UnitDelay  InitialCondition=false  SampleTime=0.02  HasFrameUpgradeWarning=on
  Perception Valid Delay : UnitDelay  InitialCondition=false  SampleTime=0.02  HasFrameUpgradeWarning=on
  Pose To Robot Transform : MATLAB Function  TreatAsAtomicUnit=on
  Robot Kinova : robotsim3dlib/Simulation 3D Robot  Priority=2  actorInputType=RigidBodyTree Object  RigidBodyTree=gen3  ActorName=Ro6Kinova  existActorChekBox=off  initialTrans=[0 0 0]  initialRot=[0 0 0]  initialConfig=qStow  EndEffector=ToolTip  eeOffsetInpChekBox=off  eeTargetTrans=[-0.04 0 0.245]  eeTargetRot=[0 1.2217 3.1416]  enableRegionGraspChekBox=on  regionGraspInpChekBox=on  eeTargTransDiff=[0.2 0.2 0.2]  eeTargRotDiff=[0 0 0]  inpConfEnbVal=on  inpGraspEnbVal=on  inpTransEnbVal=on  outConfEnbVal=on  outGraspEnbVal=on  outTransEnbVal=off  SampleTime=0.02  ActorType=SimulinkVehicle  ID=C  aMode=6  ActorTag=Ro6Kinova  Mesh=RigidBodyTree
  Robot Out Unused 1 : Terminator
  Robot Out Unused 2 : Terminator
  Robot Pack : MATLAB Function  TreatAsAtomicUnit=on
  RobotTaskFSM : Stateflow chart  TreatAsAtomicUnit=on
  Scan Done Delay : UnitDelay  InitialCondition=false  SampleTime=0.02  HasFrameUpgradeWarning=on
  Sense Bus Delay : UnitDelay  InitialCondition=zeros(1,8)  SampleTime=0.02  HasFrameUpgradeWarning=on
  Target Actor : Constant  Value=uint8('TargetBox')  OutDataTypeStr=uint8
  Target Actor uint8 : DataTypeConversion  OutDataTypeStr=uint8  SaturateOnIntegerOverflow=off  RndMeth=Floor
  Term_Differential_Drive_Kinematics_2 : Terminator
  Term_RobotTaskFSM_7 : Terminator
  Term_RobotTaskFSM_8 : Terminator
  Velocity Split : Demux  Outputs=2
  Pose : Outport
  Pack : Outport  Port=2
  Lift : Outport  Port=3
  State : Outport  Port=4
  wires:
  Navigation Arm Controller/3 -> AtGoal Delay/1
  AtGoal Delay/1 -> RobotTaskFSM/1(AtGoal)
  Navigation Arm Controller/4 -> ArmDone Delay/1
  ArmDone Delay/1 -> RobotTaskFSM/2(ArmDone)
  Navigation Arm Controller/5 -> Arm Fault Delay/1
  Arm Fault Delay/1 -> RobotTaskFSM/8(ArmFault)
  Navigation Arm Controller/6 -> Grasped Delay/1
  Grasped Delay/1 -> RobotTaskFSM/7(IsTargetGrasped), Navigation Arm Controller/8
  Navigation Arm Controller/16 -> Perception Valid Delay/1
  Perception Valid Delay/1 -> RobotTaskFSM/3(PerceptionValid)
  Navigation Arm Controller/17 -> More Boxes Delay/1
  More Boxes Delay/1 -> RobotTaskFSM/9(MoreBoxes)
  Navigation Arm Controller/18 -> Scan Done Delay/1
  Scan Done Delay/1 -> RobotTaskFSM/10(ScanDone)
  Navigation Arm Controller/19 -> Finish Delay/1
  Finish Delay/1 -> RobotTaskFSM/11(Finish)
  Navigation Arm Controller/20 -> Need Home Delay/1
  Need Home Delay/1 -> RobotTaskFSM/12(NeedHome)
  Box Coord Zero 1/1 -> RobotTaskFSM/4(BoxX)
  Box Coord Zero 2/1 -> RobotTaskFSM/5(BoxY)
  Box Coord Zero 3/1 -> RobotTaskFSM/6(BoxZ)
  RobotTaskFSM/1(TaskState) -> Navigation Arm Controller/1, State/1
  RobotTaskFSM/2(GoalX) -> Navigation Arm Controller/2
  RobotTaskFSM/3(GoalY) -> Navigation Arm Controller/3
  RobotTaskFSM/4(IKTargetX) -> Navigation Arm Controller/4
  RobotTaskFSM/5(IKTargetY) -> Navigation Arm Controller/5
  RobotTaskFSM/6(IKTargetZ) -> Navigation Arm Controller/6
  EstPose/1 -> Navigation Arm Controller/7
  SenseBus/1 -> Sense Bus Delay/1
  Sense Bus Delay/1 -> Navigation Arm Controller/10
  CamBus/1 -> Cam Bus Delay/1
  Cam Bus Delay/1 -> Navigation Arm Controller/11
  Base Pose Delay/1 -> Navigation Arm Controller/12, Pose/1, Pose To Robot Transform/1(pose)
  Navigation Arm Controller/8 -> Idx Select/1(c2), Robot Pack/4(c2)
  Idx Select/1(idx) -> Idx Delay/1
  Idx Delay/1 -> Box Meas Pick/2(idx)
  Pool/1 -> Box Meas Pick/1(pool)
  Box Meas Pick/1(y) -> Navigation Arm Controller/9
  Navigation Arm Controller/7 -> Robot Pack/1(c)
  Navigation Arm Controller/10 -> Robot Pack/2(r)
  Navigation Arm Controller/13 -> Robot Pack/3(d)
  Robot Pack/1(y) -> Pack/1
  Navigation Arm Controller/2 -> Lift Select/1(q), Robot Kinova/1
  Lift Select/1(y) -> Lift/1
  Navigation Arm Controller/9 -> Ctl Unused 9/1
  Navigation Arm Controller/11 -> Ctl Unused 11/1
  Navigation Arm Controller/12 -> Ctl Unused 12/1
  Navigation Arm Controller/14 -> Ctl Unused 14/1
  Navigation Arm Controller/15 -> Ctl Unused 15/1
  Navigation Arm Controller/1 -> Velocity Split/1
  Velocity Split/1 -> Differential Drive Kinematics/1
  Velocity Split/2 -> Differential Drive Kinematics/2
  Differential Drive Kinematics/1 -> Base Pose Delay/1
  Target Actor/1 -> Target Actor uint8/1
  Pose To Robot Transform/1(translation) -> Robot Kinova/2
  Pose To Robot Transform/2(rotation) -> Robot Kinova/3
  Target Actor uint8/1 -> Robot Kinova/4
  Native Grasp Off/1 -> Robot Kinova/5
  Grasp Translation/1 -> Robot Kinova/6
  Grasp Rotation/1 -> Robot Kinova/7
  Robot Kinova/1 -> Robot Out Unused 1/1
  Robot Kinova/2 -> Robot Out Unused 2/1
  Differential Drive Kinematics/2 -> Term_Differential_Drive_Kinematics_2/1
  RobotTaskFSM/7(GraspCmd) -> Term_RobotTaskFSM_7/1
  RobotTaskFSM/8(PlaceCmd) -> Term_RobotTaskFSM_8/1

== stateflow chart WarehouseFleetSim/Robot 1/RobotTaskFSM ==
  settings: updateMethod=DISCRETE  sampleTime=0.02
  state IDLE
    en: TaskState=uint8(0); GoalX=-20.0000; GoalY=7.3000; GraspCmd=false; PlaceCmd=false;
  state NAV_TO_STAGING
    en: TaskState=uint8(1); GoalX=15.5000; GoalY=46.0556; GraspCmd=false; PlaceCmd=false;
  state DOCK_SHELF
    en: TaskState=uint8(10); GoalX=14.1900; GoalY=46.0556; IKTargetX=BoxX; IKTargetY=BoxY; IKTargetZ=BoxZ; GraspCmd=false; PlaceCmd=false;
  state ARM_EXTEND
    en: TaskState=uint8(2); IKTargetX=BoxX; IKTargetY=BoxY; IKTargetZ=BoxZ; GraspCmd=false;
  state GRASP
    en: TaskState=uint8(3); GraspCmd=true; PlaceCmd=false;
  state ARM_RETRACT
    en: TaskState=uint8(4); GraspCmd=true; PlaceCmd=false;
  state NAV_TO_TABLE
    en: TaskState=uint8(5); GoalX=18.5000; GoalY=65.1000; GraspCmd=true;
  state ARM_PLACE
    en: TaskState=uint8(6); IKTargetX=18.5000; IKTargetY=65.9700; IKTargetZ=1.0700; GraspCmd=true;
  state RELEASE
    en: TaskState=uint8(8); GraspCmd=false; PlaceCmd=true;
  state ARM_STOW
    en: TaskState=uint8(9); GraspCmd=false; PlaceCmd=false;
  state RETURN_HOME
    en: TaskState=uint8(7); GoalX=-20.0000; GoalY=7.3000; GraspCmd=false;
  state FAULT_HOLD
    en: TaskState=uint8(11); GraspCmd=false; PlaceCmd=false;
  state MISSION_DONE
    en: TaskState=uint8(12); GoalX=-20.0000; GoalY=7.3000; GraspCmd=false; PlaceCmd=false;
  NAV_TO_STAGING -> IDLE [order 2] : [AtGoal && ScanDone && ~PerceptionValid]
  RETURN_HOME -> IDLE : [AtGoal || MoreBoxes]
  (default) -> IDLE
  GRASP -> ARM_RETRACT [order 2] : [ArmDone && IsTargetGrasped]
  DOCK_SHELF -> FAULT_HOLD [order 2] : [ArmFault]
  ARM_EXTEND -> FAULT_HOLD [order 1] : [ArmFault]
  GRASP -> FAULT_HOLD [order 1] : [ArmFault]
  IDLE -> NAV_TO_STAGING [order 1] : after(1,sec)[MoreBoxes]
  NAV_TO_STAGING -> DOCK_SHELF [order 1] : [AtGoal && ScanDone && PerceptionValid]
  DOCK_SHELF -> ARM_EXTEND [order 1] : [AtGoal && ArmDone]
  ARM_EXTEND -> GRASP [order 2] : [ArmDone]
  IDLE -> MISSION_DONE [order 3] : after(2,sec)[~MoreBoxes && Finish && ~NeedHome]
  IDLE -> RETURN_HOME [order 2] : after(1,sec)[~MoreBoxes && NeedHome]
  FAULT_HOLD -> ARM_RETRACT [order 1] : [~ArmFault && IsTargetGrasped]
  ARM_RETRACT -> NAV_TO_TABLE [order 2] : [ArmDone]
  ARM_STOW -> RETURN_HOME : [ArmDone]
  NAV_TO_TABLE -> ARM_PLACE : [AtGoal]
  ARM_PLACE -> FAULT_HOLD [order 1] : [ArmFault]
  ARM_PLACE -> RELEASE [order 2] : [ArmDone]
  FAULT_HOLD -> ARM_STOW [order 2] : [~ArmFault && ~IsTargetGrasped]
  RELEASE -> ARM_STOW [order 1] : [~IsTargetGrasped]
  RELEASE -> ARM_STOW [order 2] : after(1,sec)
  ARM_RETRACT -> FAULT_HOLD [order 1] : [ArmFault]
  data: AtGoal input boolean; ArmDone input boolean; PerceptionValid input boolean; BoxX input double; BoxY input double; BoxZ input double; IsTargetGrasped input boolean; ArmFault input boolean; MoreBoxes input boolean; ScanDone input boolean; Finish input boolean; NeedHome input boolean; TaskState output uint8; GoalX output double; GoalY output double; IKTargetX output double; IKTargetY output double; IKTargetZ output double; GraspCmd output boolean; PlaceCmd output boolean

== matlab function WarehouseFleetSim/Robot 1/Box Meas Pick ==
  data: pool input; y output; idx input
function y = fcn(pool,idx)
y = zeros(1,9); i = round(idx);
if i>=1 && i<=54, y(1:3) = pool(3*i-2:3*i); end

== matlab function WarehouseFleetSim/Robot 1/Robot Pack ==
  data: c input; y output; r input; d input; c2 input
function y = fcn(c,r,d,c2)
y = [c r double(d) c2(1)];

== matlab function WarehouseFleetSim/Robot 1/Lift Select ==
  data: q input; y output
function y = fcn(q)
y = q(1);

== matlab function WarehouseFleetSim/Robot 1/Pose To Robot Transform ==
  data: pose input; translation output; rotation output
function [translation,rotation] = fcn(pose)
translation = [pose(1), pose(2), 0];
rotation = [pose(3), 0, 0];

== stateflow chart WarehouseFleetSim/Robot 2/RobotTaskFSM ==
  settings: updateMethod=DISCRETE  sampleTime=0.02
  state IDLE
    en: TaskState=uint8(0); GoalX=-20.0000; GoalY=3.6000; GraspCmd=false; PlaceCmd=false;
  state NAV_TO_STAGING
    en: TaskState=uint8(1); GoalX=15.5000; GoalY=46.0556; GraspCmd=false; PlaceCmd=false;
  state DOCK_SHELF
    en: TaskState=uint8(10); GoalX=14.1900; GoalY=46.0556; IKTargetX=BoxX; IKTargetY=BoxY; IKTargetZ=BoxZ; GraspCmd=false; PlaceCmd=false;
  state ARM_EXTEND
    en: TaskState=uint8(2); IKTargetX=BoxX; IKTargetY=BoxY; IKTargetZ=BoxZ; GraspCmd=false;
  state GRASP
    en: TaskState=uint8(3); GraspCmd=true; PlaceCmd=false;
  state ARM_RETRACT
    en: TaskState=uint8(4); GraspCmd=true; PlaceCmd=false;
  state NAV_TO_TABLE
    en: TaskState=uint8(5); GoalX=18.5000; GoalY=65.1000; GraspCmd=true;
  state ARM_PLACE
    en: TaskState=uint8(6); IKTargetX=18.5000; IKTargetY=65.9700; IKTargetZ=1.0700; GraspCmd=true;
  state RELEASE
    en: TaskState=uint8(8); GraspCmd=false; PlaceCmd=true;
  state ARM_STOW
    en: TaskState=uint8(9); GraspCmd=false; PlaceCmd=false;
  state RETURN_HOME
    en: TaskState=uint8(7); GoalX=-20.0000; GoalY=3.6000; GraspCmd=false;
  state FAULT_HOLD
    en: TaskState=uint8(11); GraspCmd=false; PlaceCmd=false;
  state MISSION_DONE
    en: TaskState=uint8(12); GoalX=-20.0000; GoalY=3.6000; GraspCmd=false; PlaceCmd=false;
  NAV_TO_STAGING -> IDLE [order 2] : [AtGoal && ScanDone && ~PerceptionValid]
  RETURN_HOME -> IDLE : [AtGoal || MoreBoxes]
  (default) -> IDLE
  GRASP -> ARM_RETRACT [order 2] : [ArmDone && IsTargetGrasped]
  DOCK_SHELF -> FAULT_HOLD [order 2] : [ArmFault]
  ARM_EXTEND -> FAULT_HOLD [order 1] : [ArmFault]
  GRASP -> FAULT_HOLD [order 1] : [ArmFault]
  IDLE -> NAV_TO_STAGING [order 1] : after(1,sec)[MoreBoxes]
  NAV_TO_STAGING -> DOCK_SHELF [order 1] : [AtGoal && ScanDone && PerceptionValid]
  DOCK_SHELF -> ARM_EXTEND [order 1] : [AtGoal && ArmDone]
  ARM_EXTEND -> GRASP [order 2] : [ArmDone]
  IDLE -> MISSION_DONE [order 3] : after(2,sec)[~MoreBoxes && Finish && ~NeedHome]
  IDLE -> RETURN_HOME [order 2] : after(1,sec)[~MoreBoxes && NeedHome]
  FAULT_HOLD -> ARM_RETRACT [order 1] : [~ArmFault && IsTargetGrasped]
  ARM_RETRACT -> NAV_TO_TABLE [order 2] : [ArmDone]
  ARM_STOW -> RETURN_HOME : [ArmDone]
  NAV_TO_TABLE -> ARM_PLACE : [AtGoal]
  ARM_PLACE -> FAULT_HOLD [order 1] : [ArmFault]
  ARM_PLACE -> RELEASE [order 2] : [ArmDone]
  FAULT_HOLD -> ARM_STOW [order 2] : [~ArmFault && ~IsTargetGrasped]
  RELEASE -> ARM_STOW [order 1] : [~IsTargetGrasped]
  RELEASE -> ARM_STOW [order 2] : after(1,sec)
  ARM_RETRACT -> FAULT_HOLD [order 1] : [ArmFault]
  data: AtGoal input boolean; ArmDone input boolean; PerceptionValid input boolean; BoxX input double; BoxY input double; BoxZ input double; IsTargetGrasped input boolean; ArmFault input boolean; MoreBoxes input boolean; ScanDone input boolean; Finish input boolean; NeedHome input boolean; TaskState output uint8; GoalX output double; GoalY output double; IKTargetX output double; IKTargetY output double; IKTargetZ output double; GraspCmd output boolean; PlaceCmd output boolean

== matlab function WarehouseFleetSim/Robot 2/Idx Select ==
  data: c2 input; idx output
function idx = fcn(c2)
idx = c2(1);

== matlab function WarehouseFleetSim/Robot 2/Box Meas Pick ==
  data: pool input; y output; idx input
function y = fcn(pool,idx)
y = zeros(1,9); i = round(idx);
if i>=1 && i<=54, y(1:3) = pool(3*i-2:3*i); end

== matlab function WarehouseFleetSim/Robot 2/Robot Pack ==
  data: c input; y output; r input; d input; c2 input
function y = fcn(c,r,d,c2)
y = [c r double(d) c2(1)];

== matlab function WarehouseFleetSim/Robot 2/Lift Select ==
  data: q input; y output
function y = fcn(q)
y = q(1);

== matlab function WarehouseFleetSim/Robot 2/Pose To Robot Transform ==
  data: pose input; translation output; rotation output
function [translation,rotation] = fcn(pose)
translation = [pose(1), pose(2), 0];
rotation = [pose(3), 0, 0];

== stateflow chart WarehouseFleetSim/Robot 3/RobotTaskFSM ==
  settings: updateMethod=DISCRETE  sampleTime=0.02
  state IDLE
    en: TaskState=uint8(0); GoalX=-20.0000; GoalY=11.0000; GraspCmd=false; PlaceCmd=false;
  state NAV_TO_STAGING
    en: TaskState=uint8(1); GoalX=15.5000; GoalY=46.0556; GraspCmd=false; PlaceCmd=false;
  state DOCK_SHELF
    en: TaskState=uint8(10); GoalX=14.1900; GoalY=46.0556; IKTargetX=BoxX; IKTargetY=BoxY; IKTargetZ=BoxZ; GraspCmd=false; PlaceCmd=false;
  state ARM_EXTEND
    en: TaskState=uint8(2); IKTargetX=BoxX; IKTargetY=BoxY; IKTargetZ=BoxZ; GraspCmd=false;
  state GRASP
    en: TaskState=uint8(3); GraspCmd=true; PlaceCmd=false;
  state ARM_RETRACT
    en: TaskState=uint8(4); GraspCmd=true; PlaceCmd=false;
  state NAV_TO_TABLE
    en: TaskState=uint8(5); GoalX=18.5000; GoalY=65.1000; GraspCmd=true;
  state ARM_PLACE
    en: TaskState=uint8(6); IKTargetX=18.5000; IKTargetY=65.9700; IKTargetZ=1.0700; GraspCmd=true;
  state RELEASE
    en: TaskState=uint8(8); GraspCmd=false; PlaceCmd=true;
  state ARM_STOW
    en: TaskState=uint8(9); GraspCmd=false; PlaceCmd=false;
  state RETURN_HOME
    en: TaskState=uint8(7); GoalX=-20.0000; GoalY=11.0000; GraspCmd=false;
  state FAULT_HOLD
    en: TaskState=uint8(11); GraspCmd=false; PlaceCmd=false;
  state MISSION_DONE
    en: TaskState=uint8(12); GoalX=-20.0000; GoalY=11.0000; GraspCmd=false; PlaceCmd=false;
  NAV_TO_STAGING -> IDLE [order 2] : [AtGoal && ScanDone && ~PerceptionValid]
  RETURN_HOME -> IDLE : [AtGoal || MoreBoxes]
  (default) -> IDLE
  GRASP -> ARM_RETRACT [order 2] : [ArmDone && IsTargetGrasped]
  DOCK_SHELF -> FAULT_HOLD [order 2] : [ArmFault]
  ARM_EXTEND -> FAULT_HOLD [order 1] : [ArmFault]
  GRASP -> FAULT_HOLD [order 1] : [ArmFault]
  IDLE -> NAV_TO_STAGING [order 1] : after(1,sec)[MoreBoxes]
  NAV_TO_STAGING -> DOCK_SHELF [order 1] : [AtGoal && ScanDone && PerceptionValid]
  DOCK_SHELF -> ARM_EXTEND [order 1] : [AtGoal && ArmDone]
  ARM_EXTEND -> GRASP [order 2] : [ArmDone]
  IDLE -> MISSION_DONE [order 3] : after(2,sec)[~MoreBoxes && Finish && ~NeedHome]
  IDLE -> RETURN_HOME [order 2] : after(1,sec)[~MoreBoxes && NeedHome]
  FAULT_HOLD -> ARM_RETRACT [order 1] : [~ArmFault && IsTargetGrasped]
  ARM_RETRACT -> NAV_TO_TABLE [order 2] : [ArmDone]
  ARM_STOW -> RETURN_HOME : [ArmDone]
  NAV_TO_TABLE -> ARM_PLACE : [AtGoal]
  ARM_PLACE -> FAULT_HOLD [order 1] : [ArmFault]
  ARM_PLACE -> RELEASE [order 2] : [ArmDone]
  FAULT_HOLD -> ARM_STOW [order 2] : [~ArmFault && ~IsTargetGrasped]
  RELEASE -> ARM_STOW [order 1] : [~IsTargetGrasped]
  RELEASE -> ARM_STOW [order 2] : after(1,sec)
  ARM_RETRACT -> FAULT_HOLD [order 1] : [ArmFault]
  data: AtGoal input boolean; ArmDone input boolean; PerceptionValid input boolean; BoxX input double; BoxY input double; BoxZ input double; IsTargetGrasped input boolean; ArmFault input boolean; MoreBoxes input boolean; ScanDone input boolean; Finish input boolean; NeedHome input boolean; TaskState output uint8; GoalX output double; GoalY output double; IKTargetX output double; IKTargetY output double; IKTargetZ output double; GraspCmd output boolean; PlaceCmd output boolean

== matlab function WarehouseFleetSim/Robot 3/Idx Select ==
  data: c2 input; idx output
function idx = fcn(c2)
idx = c2(1);

== matlab function WarehouseFleetSim/Robot 3/Box Meas Pick ==
  data: pool input; y output; idx input
function y = fcn(pool,idx)
y = zeros(1,9); i = round(idx);
if i>=1 && i<=54, y(1:3) = pool(3*i-2:3*i); end

== matlab function WarehouseFleetSim/Robot 3/Robot Pack ==
  data: c input; y output; r input; d input; c2 input
function y = fcn(c,r,d,c2)
y = [c r double(d) c2(1)];

== matlab function WarehouseFleetSim/Robot 3/Lift Select ==
  data: q input; y output
function y = fcn(q)
y = q(1);

== matlab function WarehouseFleetSim/Robot 3/Pose To Robot Transform ==
  data: pose input; translation output; rotation output
function [translation,rotation] = fcn(pose)
translation = [pose(1), pose(2), 0];
rotation = [pose(3), 0, 0];

== stateflow chart WarehouseFleetSim/Robot 4/RobotTaskFSM ==
  settings: updateMethod=DISCRETE  sampleTime=0.02
  state IDLE
    en: TaskState=uint8(0); GoalX=-24.5000; GoalY=3.6000; GraspCmd=false; PlaceCmd=false;
  state NAV_TO_STAGING
    en: TaskState=uint8(1); GoalX=15.5000; GoalY=46.0556; GraspCmd=false; PlaceCmd=false;
  state DOCK_SHELF
    en: TaskState=uint8(10); GoalX=14.1900; GoalY=46.0556; IKTargetX=BoxX; IKTargetY=BoxY; IKTargetZ=BoxZ; GraspCmd=false; PlaceCmd=false;
  state ARM_EXTEND
    en: TaskState=uint8(2); IKTargetX=BoxX; IKTargetY=BoxY; IKTargetZ=BoxZ; GraspCmd=false;
  state GRASP
    en: TaskState=uint8(3); GraspCmd=true; PlaceCmd=false;
  state ARM_RETRACT
    en: TaskState=uint8(4); GraspCmd=true; PlaceCmd=false;
  state NAV_TO_TABLE
    en: TaskState=uint8(5); GoalX=18.5000; GoalY=65.1000; GraspCmd=true;
  state ARM_PLACE
    en: TaskState=uint8(6); IKTargetX=18.5000; IKTargetY=65.9700; IKTargetZ=1.0700; GraspCmd=true;
  state RELEASE
    en: TaskState=uint8(8); GraspCmd=false; PlaceCmd=true;
  state ARM_STOW
    en: TaskState=uint8(9); GraspCmd=false; PlaceCmd=false;
  state RETURN_HOME
    en: TaskState=uint8(7); GoalX=-24.5000; GoalY=3.6000; GraspCmd=false;
  state FAULT_HOLD
    en: TaskState=uint8(11); GraspCmd=false; PlaceCmd=false;
  state MISSION_DONE
    en: TaskState=uint8(12); GoalX=-24.5000; GoalY=3.6000; GraspCmd=false; PlaceCmd=false;
  NAV_TO_STAGING -> IDLE [order 2] : [AtGoal && ScanDone && ~PerceptionValid]
  RETURN_HOME -> IDLE : [AtGoal || MoreBoxes]
  (default) -> IDLE
  GRASP -> ARM_RETRACT [order 2] : [ArmDone && IsTargetGrasped]
  DOCK_SHELF -> FAULT_HOLD [order 2] : [ArmFault]
  ARM_EXTEND -> FAULT_HOLD [order 1] : [ArmFault]
  GRASP -> FAULT_HOLD [order 1] : [ArmFault]
  IDLE -> NAV_TO_STAGING [order 1] : after(1,sec)[MoreBoxes]
  NAV_TO_STAGING -> DOCK_SHELF [order 1] : [AtGoal && ScanDone && PerceptionValid]
  DOCK_SHELF -> ARM_EXTEND [order 1] : [AtGoal && ArmDone]
  ARM_EXTEND -> GRASP [order 2] : [ArmDone]
  IDLE -> MISSION_DONE [order 3] : after(2,sec)[~MoreBoxes && Finish && ~NeedHome]
  IDLE -> RETURN_HOME [order 2] : after(1,sec)[~MoreBoxes && NeedHome]
  FAULT_HOLD -> ARM_RETRACT [order 1] : [~ArmFault && IsTargetGrasped]
  ARM_RETRACT -> NAV_TO_TABLE [order 2] : [ArmDone]
  ARM_STOW -> RETURN_HOME : [ArmDone]
  NAV_TO_TABLE -> ARM_PLACE : [AtGoal]
  ARM_PLACE -> FAULT_HOLD [order 1] : [ArmFault]
  ARM_PLACE -> RELEASE [order 2] : [ArmDone]
  FAULT_HOLD -> ARM_STOW [order 2] : [~ArmFault && ~IsTargetGrasped]
  RELEASE -> ARM_STOW [order 1] : [~IsTargetGrasped]
  RELEASE -> ARM_STOW [order 2] : after(1,sec)
  ARM_RETRACT -> FAULT_HOLD [order 1] : [ArmFault]
  data: AtGoal input boolean; ArmDone input boolean; PerceptionValid input boolean; BoxX input double; BoxY input double; BoxZ input double; IsTargetGrasped input boolean; ArmFault input boolean; MoreBoxes input boolean; ScanDone input boolean; Finish input boolean; NeedHome input boolean; TaskState output uint8; GoalX output double; GoalY output double; IKTargetX output double; IKTargetY output double; IKTargetZ output double; GraspCmd output boolean; PlaceCmd output boolean

== matlab function WarehouseFleetSim/Robot 4/Idx Select ==
  data: c2 input; idx output
function idx = fcn(c2)
idx = c2(1);

== matlab function WarehouseFleetSim/Robot 4/Box Meas Pick ==
  data: pool input; y output; idx input
function y = fcn(pool,idx)
y = zeros(1,9); i = round(idx);
if i>=1 && i<=54, y(1:3) = pool(3*i-2:3*i); end

== matlab function WarehouseFleetSim/Robot 4/Robot Pack ==
  data: c input; y output; r input; d input; c2 input
function y = fcn(c,r,d,c2)
y = [c r double(d) c2(1)];

== matlab function WarehouseFleetSim/Robot 4/Lift Select ==
  data: q input; y output
function y = fcn(q)
y = q(1);

== matlab function WarehouseFleetSim/Robot 4/Pose To Robot Transform ==
  data: pose input; translation output; rotation output
function [translation,rotation] = fcn(pose)
translation = [pose(1), pose(2), 0];
rotation = [pose(3), 0, 0];
